simulink model "Eight"  (R2016a)
settings: Solver=VariableStepAuto  StartTime=0.0  StopTime=100  RelTol=1e-3
undefined symbols (not defined in the file or in its folder): aWS, bWS
libraries: simulink x2
settings Model: Creator=kkhan  LastModifiedBy=kkhan

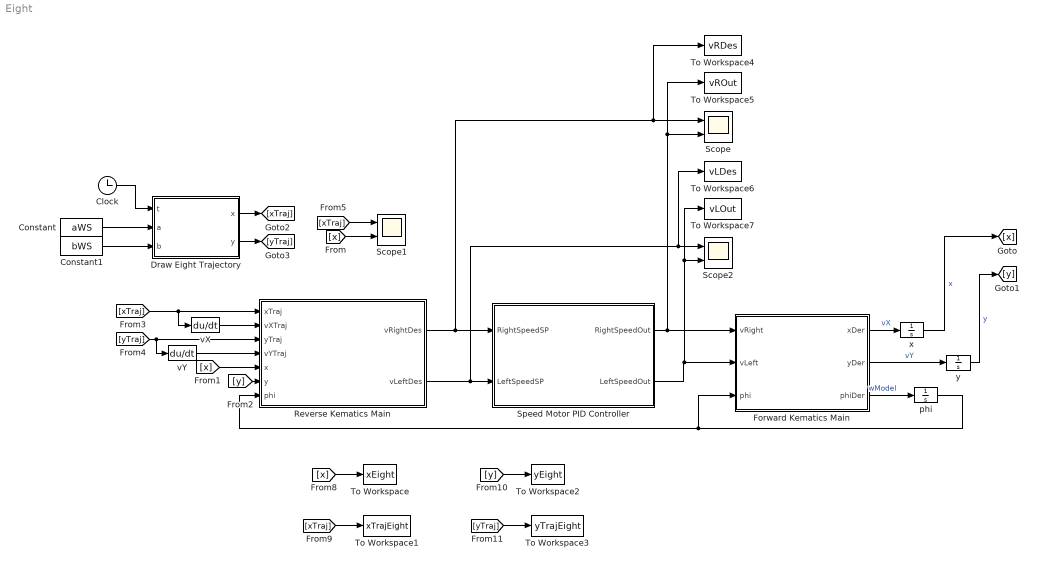
== system Eight ==
  Clock : Clock
  Constant : Constant  Value=aWS
  Constant1 : Constant  Value=bWS
  Draw Eight Trajectory : MATLAB Function  TreatAsAtomicUnit=on
  Forward Kematics Main : MATLAB Function  TreatAsAtomicUnit=on
  Reverse Kematics Main : MATLAB Function  TreatAsAtomicUnit=on
  Scope : Scope  NumInputPorts=2
  Scope1 : Scope  NumInputPorts=2
  Scope2 : Scope  NumInputPorts=2
  Speed Motor PID Controller : Subsystem  TreatAsAtomicUnit=on
  To Workspace : ToWorkspace  VariableName=xEight  SaveFormat=Timeseries  SampleTime=-1
      settings: Decimation=2
  To Workspace1 : ToWorkspace  VariableName=xTrajEight  SaveFormat=Timeseries  SampleTime=-1
      settings: Decimation=2
  To Workspace2 : ToWorkspace  VariableName=yEight  SaveFormat=Timeseries  SampleTime=-1
      settings: Decimation=2
  To Workspace3 : ToWorkspace  VariableName=yTrajEight  SaveFormat=Timeseries  SampleTime=-1
      settings: Decimation=2
  To Workspace4 : ToWorkspace  VariableName=vRDes  SaveFormat=Timeseries  SampleTime=-1
      settings: Decimation=2
  To Workspace5 : ToWorkspace  VariableName=vROut  SaveFormat=Timeseries  SampleTime=-1
      settings: Decimation=2
  To Workspace6 : ToWorkspace  VariableName=vLDes  SaveFormat=Timeseries  SampleTime=-1
      settings: Decimation=2
  To Workspace7 : ToWorkspace  VariableName=vLOut  SaveFormat=Timeseries  SampleTime=-1
      settings: Decimation=2
  phi : Integrator
  vX : Derivative
  vY : Derivative
  x : Integrator
  y : Integrator
  wires:
  Speed Motor PID Controller/2(LeftSpeedOut) -> To Workspace7/1, Scope2/2, Forward Kematics Main/2(vLeft)
  Forward Kematics Main/1(xDer) -> x/1  "vX"
  Forward Kematics Main/2(yDer) -> y/1  "vY"
  x/1 -> [x]  "x"
  y/1 -> [y]  "y"
  Forward Kematics Main/3(phiDer) -> phi/1  "wModel"
  phi/1 -> Reverse Kematics Main/7(phi), Forward Kematics Main/3(phi)
  vX/1 -> Reverse Kematics Main/2(vXTraj)
  vY/1 -> Reverse Kematics Main/4(vYTraj)
  [x] -> Scope1/2
  [x] -> Reverse Kematics Main/5(x)
  [y] -> Reverse Kematics Main/6(y)
  Draw Eight Trajectory/1(x) -> [xTraj]
  Draw Eight Trajectory/2(y) -> [yTraj]
  [xTraj] -> vX/1, Reverse Kematics Main/1(xTraj)
  [yTraj] -> vY/1, Reverse Kematics Main/3(yTraj)
  [xTraj] -> Scope1/1
  [x] -> To Workspace/1
  [xTraj] -> To Workspace1/1
  [y] -> To Workspace2/1
  [yTraj] -> To Workspace3/1
  Reverse Kematics Main/1(vRightDes) -> Speed Motor PID Controller/1(RightSpeedSP), To Workspace4/1, Scope/1
  Speed Motor PID Controller/1(RightSpeedOut) -> Forward Kematics Main/1(vRight), Scope/2, To Workspace5/1
  Reverse Kematics Main/2(vLeftDes) -> Speed Motor PID Controller/2(LeftSpeedSP), To Workspace6/1, Scope2/1
  Clock/1 -> Draw Eight Trajectory/1(t)
  Constant/1 -> Draw Eight Trajectory/2(a)
  Constant1/1 -> Draw Eight Trajectory/3(b)

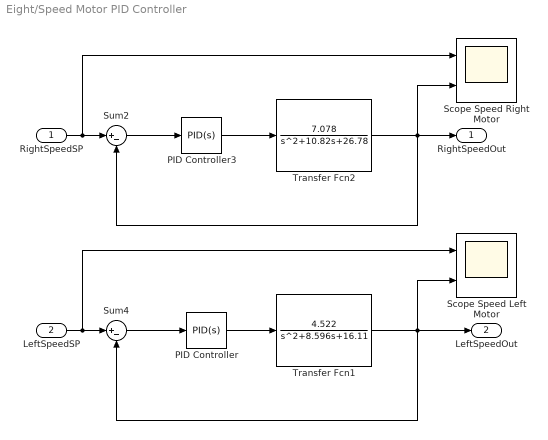
== system Eight/Speed Motor PID Controller ==
  RightSpeedSP : Inport
  LeftSpeedSP : Inport  Port=2
  PID Controller : simulink/Continuous/PID Controller  Controller=PID  TimeDomain=Continuous-time  SampleTime=-1  IntegratorMethod=Forward Euler  FilterMethod=Forward Euler  Form=Parallel  UseFilter=on  ControllerParametersSource=internal  P=17.0258243180127  I=45.6763189239245  D=1.27968580342952  N=83.9177246481862  InitialConditionSource=internal  InitialConditionForIntegrator=0  InitialConditionForFilter=0  ExternalReset=none  LimitOutput=off  UpperSaturationLimit=inf  LowerSaturationLimit=-inf  LinearizeAsGain=on  AntiWindupMode=none  Kb=1  TrackingMode=off  Kt=1  PParamMin=[]  PParamMax=[]  IParamMin=[]  IParamMax=[]  DParamMin=[]  DParamMax=[]  NParamMin=[]  NParamMax=[]  KbParamMin=[]  KbParamMax=[]  KtParamMin=[]  KtParamMax=[]  POutMin=[]  POutMax=[]  IOutMin=[]  IOutMax=[]  DOutMin=[]  DOutMax=[]  NOutMin=[]  NOutMax=[]  KbOutMin=[]  KbOutMax=[]  KtOutMin=[]  KtOutMax=[]  IntegratorOutMin=[]  IntegratorOutMax=[]  FilterOutMin=[]  FilterOutMax=[]  SumOutMin=[]  SumOutMax=[]  SumI1OutMin=[]  SumI1OutMax=[]  SumI2OutMin=[]  SumI2OutMax=[]  SumI3OutMin=[]  SumI3OutMax=[]  SumDOutMin=[]  SumDOutMax=[]  SaturationOutMin=[]  SaturationOutMax=[]  IntegratorContinuousStateAttributes=''  IntegratorStateMustResolveToSignalObject=off  IntegratorRTWStateStorageClass=Auto  FilterContinuousStateAttributes=''  FilterStateMustResolveToSignalObject=off  FilterRTWStateStorageClass=Auto  DifferentiatorICPrevScaledInput=0  DifferentiatorOutMin=[]  DifferentiatorOutMax=[]
  PID Controller3 : simulink/Continuous/PID Controller  Controller=PID  TimeDomain=Continuous-time  SampleTime=-1  IntegratorMethod=Forward Euler  FilterMethod=Forward Euler  Form=Parallel  UseFilter=on  ControllerParametersSource=internal  P=12.7137787264422  I=45.1328798006328  D=0.777904407581587  N=83.9177246481862  InitialConditionSource=internal  InitialConditionForIntegrator=0  InitialConditionForFilter=0  ExternalReset=none  LimitOutput=off  UpperSaturationLimit=inf  LowerSaturationLimit=-inf  LinearizeAsGain=on  AntiWindupMode=none  Kb=1  TrackingMode=off  Kt=1  PParamMin=[]  PParamMax=[]  IParamMin=[]  IParamMax=[]  DParamMin=[]  DParamMax=[]  NParamMin=[]  NParamMax=[]  KbParamMin=[]  KbParamMax=[]  KtParamMin=[]  KtParamMax=[]  POutMin=[]  POutMax=[]  IOutMin=[]  IOutMax=[]  DOutMin=[]  DOutMax=[]  NOutMin=[]  NOutMax=[]  KbOutMin=[]  KbOutMax=[]  KtOutMin=[]  KtOutMax=[]  IntegratorOutMin=[]  IntegratorOutMax=[]  FilterOutMin=[]  FilterOutMax=[]  SumOutMin=[]  SumOutMax=[]  SumI1OutMin=[]  SumI1OutMax=[]  SumI2OutMin=[]  SumI2OutMax=[]  SumI3OutMin=[]  SumI3OutMax=[]  SumDOutMin=[]  SumDOutMax=[]  SaturationOutMin=[]  SaturationOutMax=[]  IntegratorContinuousStateAttributes=''  IntegratorStateMustResolveToSignalObject=off  IntegratorRTWStateStorageClass=Auto  FilterContinuousStateAttributes=''  FilterStateMustResolveToSignalObject=off  FilterRTWStateStorageClass=Auto  DifferentiatorICPrevScaledInput=0  DifferentiatorOutMin=[]  DifferentiatorOutMax=[]
  Scope Speed Left Motor : Scope  NumInputPorts=2
  Scope Speed Right Motor : Scope  NumInputPorts=2
  Sum2 : Sum  Inputs=|+-
  Sum4 : Sum  Inputs=|+-
  Transfer Fcn1 : TransferFcn  Numerator=[4.522]  Denominator=[1 8.596 16.11]
  Transfer Fcn2 : TransferFcn  Numerator=[7.078]  Denominator=[1 10.82 26.78]
  RightSpeedOut : Outport
  LeftSpeedOut : Outport  Port=2
  wires:
  RightSpeedSP/1 -> Scope Speed Right Motor/1, Sum2/1
  Transfer Fcn2/1 -> Scope Speed Right Motor/2, RightSpeedOut/1, Sum2/2
  Sum2/1 -> PID Controller3/1
  PID Controller3/1 -> Transfer Fcn2/1
  LeftSpeedSP/1 -> Scope Speed Left Motor/1, Sum4/1
  Transfer Fcn1/1 -> Scope Speed Left Motor/2, LeftSpeedOut/1, Sum4/2
  Sum4/1 -> PID Controller/1
  PID Controller/1 -> Transfer Fcn1/1

== matlab function Eight/Forward Kematics Main ==
  data: vRight input; xDer output; vLeft input; yDer output; phiDer output; phi input
function [xDer,yDer,phiDer] = forward(vRight, vLeft, phi)
%#codegen
%Thong so mo hinh
lWheel = 8;
c = 4;
%Input la van toc [cm/s]
vModel = (vRight + vLeft)/2;
%Van toc goc nay la cua mo hinh
wModel = (vRight - vLeft)/(2*lWheel);

vectorMatrix = [cos(phi), -c*sin(phi);
            sin(phi), c*cos(phi);
            0, 1];
velMatrix = [vModel;wModel];

posMatrix = vectorMatrix*velMatrix;

xDer = posMatrix(1);
yDer = posMatrix(2);
phiDer = posMatrix(3);

== matlab function Eight/Reverse Kematics Main ==
  data: xTraj input; vXTraj input; yTraj input; vYTraj input; x input; y input; vRightDes output; vLeftDes output; phi input
function [vRightDes,vLeftDes] = fcn(xTraj,vXTraj,yTraj,vYTraj,x,y,phi)
%#codegen
L = 16;
c = 4;
lx = 22;
ly = 18;
kx = 1;
ky = 1;
%Input la toa do x, y
%Tu do dao ham se ra van toc dai [cm/s]
stateMatrix = [cos(phi), sin(phi);
               (-1/c)*sin(phi), (1/c)*cos(phi)];
velMatrix = stateMatrix*[vXTraj + lx*tanh((kx/lx)*(xTraj-x));
                         vYTraj + ly*tanh((ky/ly)*(yTraj-y))];

M = [1, L/2; 1, -L/2];
velRLMatrix = M*velMatrix;

vRightDes = velRLMatrix(1);
vLeftDes = velRLMatrix(2);

== matlab function Eight/Draw Eight Trajectory ==
  data: x output; y output; t input; a input; b input
function [x,y] = eight(t,a,b)
%#codegen
w = pi/16;
x = a*sin(w*t);
y = (b/2)*sin(2*w*t);
